simulink model "PV_Source_shading"  (R2025b)
settings: Solver=FixedStepDiscrete  StartTime=0.0  StopTime=0.5  FixedStep=Ts  RelTol=1e-3
InitFcn:
  | Ts = 1e-06;
libraries: spsSeriesRLCBranchLib x4, spsDiodeLib x3, spsPVArrayLib x2, spsVoltageMeasurementLib x2, simulink x1, spsCurrentMeasurementLib x1, spsIdealSwitchLib x1, spsDCVoltageSourceLib x1, spspowerguiLib x1
settings Model: Creator=JESHNU PRANAV  LastModifiedBy=JESHNU PRANAV
settings SolverCC: AutoInsertRateTranBlk=on

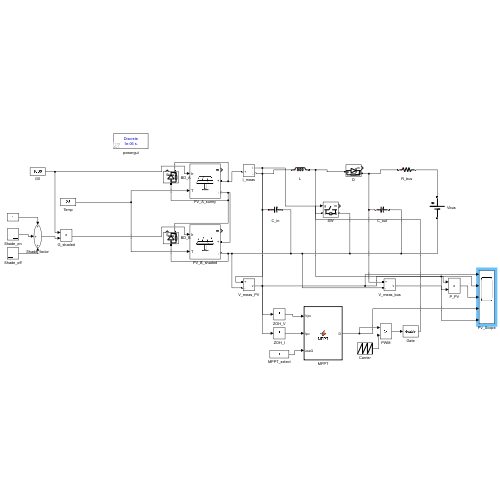
[thumbnail: Simulink's stored preview of the top-level diagram]
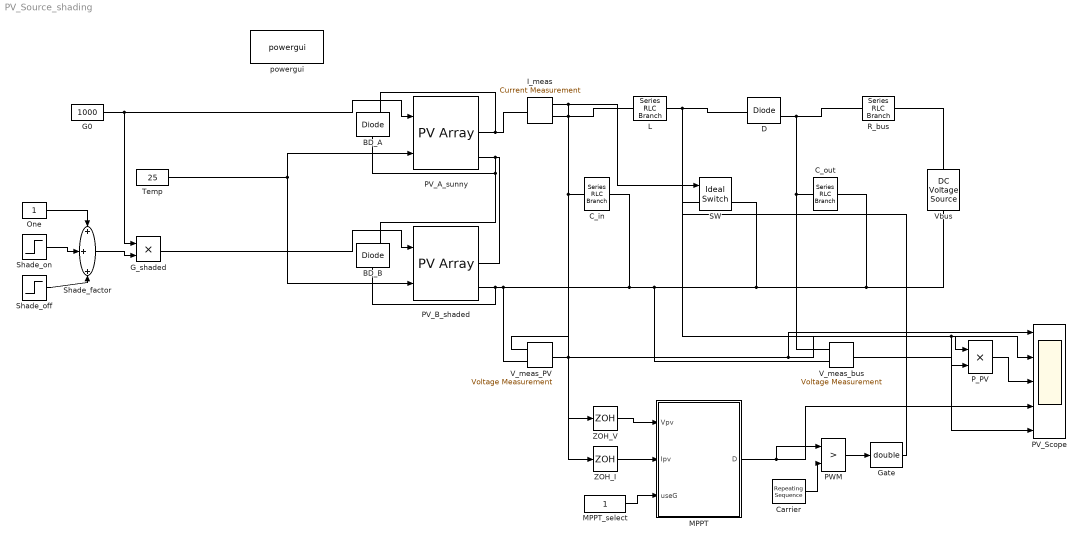
== system PV_Source_shading ==
  BD_A : spsDiodeLib/Diode  Ron=0.001  Lon=0  Vf=0.8  IC=0  UseSnubber=0  Rs=500  Cs=250e-9  Measurements=on
  BD_B : spsDiodeLib/Diode  Ron=0.001  Lon=0  Vf=0.8  IC=0  UseSnubber=0  Rs=500  Cs=250e-9  Measurements=on
  C_in : spsSeriesRLCBranchLib/Series RLC Branch  LConnTagsString=__new0  RConnTagsString=__new0  BranchType=C  Resistance=1  Inductance=1e-3  SetiL0=off  InitialCurrent=0  Capacitance=270e-6  Setx0=off  InitialVoltage=0  Measurements=None
  C_out : spsSeriesRLCBranchLib/Series RLC Branch  LConnTagsString=__new0  RConnTagsString=__new0  BranchType=C  Resistance=1  Inductance=1e-3  SetiL0=off  InitialCurrent=0  Capacitance=270e-6  Setx0=off  InitialVoltage=0  Measurements=None
  Carrier : simulink/Sources/Repeating Sequence  rep_seq_t=[0 5e-05]  rep_seq_y=[0 1]
  D : spsDiodeLib/Diode  Ron=0.001  Lon=0  Vf=0.8  IC=0  UseSnubber=0  Rs=500  Cs=250e-9  Measurements=on
  G0 : Constant  Value=1000
  G_shaded : Product
  Gate : DataTypeConversion  OutDataTypeStr=double  SaturateOnIntegerOverflow=off  RndMeth=Floor
  I_meas : spsCurrentMeasurementLib/Current Measurement  PhasorSimulation=off  OutputType=Complex  PSBequivalent=0
  L : spsSeriesRLCBranchLib/Series RLC Branch  LConnTagsString=__new0  RConnTagsString=__new0  BranchType=L  Resistance=1  Inductance=0.30e-3  SetiL0=off  InitialCurrent=0  Capacitance=1e-6  Setx0=off  InitialVoltage=0  Measurements=None
  MPPT : MATLAB Function  TreatAsAtomicUnit=on
  MPPT_select : Constant
  One : Constant
  PV_A_sunny : spsPVArrayLib/PV Array  Npar=8  Nser=4  PlotType=array @ 1000 W/m2 & specified temperatures  S_vec="[ 1000  500  100 ]"  Temp_C_vec="[ 45 25  ]"  ModuleName=User-defined  PlotWhenSelected=off  Pm=400  Ncell=72  Voc=48  Isc=10.5  Vm=40  Im=10  beta_Voc_pc=-0.36099  alpha_Isc_pc=0.102  beta_Voc=-0.17328  alpha_Isc=0.01071  IL=10.576  I0=3.9433e-10  nI=1.0809  Rsh=821.7644  Rs=0.20021  RobustModel=off  RobustCellTemperature=313.3991  BAL=on  Tc=1e-6  Tfilter=5e-5
  PV_B_shaded : spsPVArrayLib/PV Array  Npar=8  Nser=2  PlotType=array @ 1000 W/m2 & specified temperatures  S_vec="[ 1000  500  100 ]"  Temp_C_vec="[ 45 25  ]"  ModuleName=User-defined  PlotWhenSelected=off  Pm=400  Ncell=72  Voc=48  Isc=10.5  Vm=40  Im=10  beta_Voc_pc=-0.36099  alpha_Isc_pc=0.102  beta_Voc=-0.17328  alpha_Isc=0.01071  IL=10.576  I0=3.9433e-10  nI=1.0809  Rsh=821.7644  Rs=0.20021  RobustModel=off  RobustCellTemperature=313.3991  BAL=on  Tc=1e-6  Tfilter=5e-5
  PV_Scope : Scope  NumInputPorts=5
      settings: ActiveDisplayYMinimum=-928.47453257571487  ActiveDisplayYMaximum=10931.455878760957  DataLoggingDecimation=20  DataLoggingVariableName=pvdata
  PWM : RelationalOperator  Operator=>  OutDataTypeStr=boolean  RndMeth=Simplest  InputSameDT=off
  P_PV : Product
  R_bus : spsSeriesRLCBranchLib/Series RLC Branch  LConnTagsString=__new0  RConnTagsString=__new0  BranchType=R  Resistance=0.1  Inductance=1e-3  SetiL0=off  InitialCurrent=0  Capacitance=1e-6  Setx0=off  InitialVoltage=0  Measurements=None
  SW : spsIdealSwitchLib/Ideal Switch  Ron=0.001  Lon=0  IC=0  Rs=1e5  Cs=inf  Measurements=on
  Shade_factor : Sum  Inputs=+++
  Shade_off : Step  Time=0.35  After=0.7  SampleTime=0
  Shade_on : Step  Time=0.15  After=-0.7  SampleTime=0
  Temp : Constant  Value=25
  V_meas_PV : spsVoltageMeasurementLib/Voltage Measurement  PhasorSimulation=off  OutputType=Complex  PSBequivalent=0
  V_meas_bus : spsVoltageMeasurementLib/Voltage Measurement  PhasorSimulation=off  OutputType=Complex  PSBequivalent=0
  Vbus : spsDCVoltageSourceLib/DC Voltage Source  Amplitude=400  Measurements=None
  ZOH_I : ZeroOrderHold  SampleTime=0.0001
  ZOH_V : ZeroOrderHold  SampleTime=0.0001
  powergui : spspowerguiLib/powergui  Priority=1  SimulationMode=Discrete  SampleTime=Ts  frequency=60  Iterations=50  frequencyindice=0  Pbase=100e6  ErrMax=1e-4  UnitsV=kV  UnitsW=MW  buscounter=0  FunctionMessages=off  echomessages=off  EnableUseOfTLC=off  CurrentSourceSwitches=off  DisableSnubberDevices=off  DisableRonSwitches=off  DisableVfSwitches=off  DisplayEquations=off  AutomaticDiscreteSolvers=off  SolverType=Tustin/Backward Euler (TBE)  Interpol=off  ExternalGateDelay=off  methode=off  Ts=100  x0status=blocks  SPID=on  SwTol=0  HookPort=off  NonlinearTolerance=1e-4  nMaxIteration=100  ContinueOnMaxIteration=off  RestoreLinks=warning  ResistiveCurrentMeasurement=off  Frange=[0:2:500]  Ylog=off  Xlog=on  ShowGrid=off  save=off  variable=ZData  structure=0  ZoomFFT=off  StartTime=0.0  cycles=1  DisplayStyle=1  fundamental=60  FreqAxis=off  MaxFrequency=1000  frequencyindicesteady=1  RmsSteady=1  display=off
  wires:
  One/1 -> Shade_factor/1
  Shade_on/1 -> Shade_factor/2
  Shade_off/1 -> Shade_factor/3
  G0/1 -> G_shaded/1, PV_A_sunny/1
  Shade_factor/1 -> G_shaded/2
  G_shaded/1 -> PV_B_shaded/1
  Temp/1 -> PV_A_sunny/2, PV_B_shaded/2
  V_meas_PV/1 -> P_PV/1, PV_Scope/1, ZOH_V/1
  I_meas/1 -> P_PV/2, PV_Scope/2, ZOH_I/1
  ZOH_V/1 -> MPPT/1(Vpv)
  ZOH_I/1 -> MPPT/2(Ipv)
  MPPT_select/1 -> MPPT/3(useG)
  MPPT/1(D) -> PWM/1, PV_Scope/4
  Carrier/1 -> PWM/2
  PWM/1 -> Gate/1
  Gate/1 -> SW/1
  P_PV/1 -> PV_Scope/3
  V_meas_bus/1 -> PV_Scope/5
  connections:
  I_meas/LConn1 -- PV_A_sunny/RConn1 -- BD_A/RConn1
  PV_B_shaded/RConn1 -- PV_A_sunny/RConn2 -- BD_A/LConn1 -- BD_B/RConn1
  C_in/LConn1 -- I_meas/RConn1 -- L/LConn1 -- V_meas_PV/LConn1
  SW/LConn1 -- L/RConn1 -- D/LConn1
  C_out/LConn1 -- D/RConn1 -- R_bus/LConn1 -- V_meas_bus/LConn1
  R_bus/RConn1 -- Vbus/RConn1
  BD_B/LConn1 -- PV_B_shaded/RConn2 -- C_out/RConn1 -- Vbus/LConn1 -- SW/RConn1 -- V_meas_bus/LConn2 -- C_in/RConn1 -- V_meas_PV/LConn2

== matlab function PV_Source_shading/MPPT ==
  data: Vpv input; D output; Ipv input; useG input
function D = MPPT(Vpv, Ipv, useG)
% useG = 0 : standard P&O
% useG = 1 : Global MPPT = event-triggered full scan + P&O
% Boost on a 400 V bus: Vpv = (1 - D)*400, lowering D raises Vpv.
persistent mstate Dold Vold Pold k Dbest Pbest Pref holdc Psum
if isempty(mstate)
    Vold = 0; Pold = 0; k = 0; Pbest = 0; Pref = 0; holdc = 0; Psum = 0;
    if useG > 0.5, mstate = 1; Dold = 0.70; Dbest = 0.70;
    else,          mstate = 0; Dold = 0.40; Dbest = 0.40; end
end
dD = 0.002;  P = Vpv*Ipv;

if useG < 0.5   % ---------- standard P&O ----------
    dV = Vpv - Vold;  dP = P - Pold;
    if dP == 0, D = Dold; elseif dP*dV > 0, D = Dold - dD; else, D = Dold + dD; end
    D = min(max(D, 0.05), 0.85);
    Vold = Vpv; Pold = P; Dold = D;
    return
end

% ---------- Global MPPT ----------
Dlo = 0.30; Dhi = 0.70;      % scan range: Vpv = 280 V ... 120 V
dscan = 0.025; nset = 40; navg = 10;   % 17 points x 4 ms = ~70 ms scan
if mstate == 1               % SCAN: step D, wait to settle, record power
    k = k + 1;
    if k > nset - navg, Psum = Psum + P; end
    if k >= nset
        Pm = Psum/navg;
        if Pm > Pbest, Pbest = Pm; Dbest = Dold; end
        k = 0; Psum = 0;
        D = Dold - dscan;
        if D < Dlo - 1e-9     % scan done: jump to the best (global) point
            D = Dbest; mstate = 0; Pref = Pbest; holdc = 300;
        end
    else
        D = Dold;
    end
    Vold = Vpv; Pold = P; Dold = D;
    return
end
% P&O around the global peak
dV = Vpv - Vold;  dP = P - Pold;
if dP == 0, D = Dold; elseif dP*dV > 0, D = Dold - dD; else, D = Dold + dD; end
D = min(max(D, Dlo), Dhi);
if holdc > 0
    holdc = holdc - 1;
elseif Pref > 0 && abs(P - Pref) > 0.15*Pref   % sudden change (shading) -> rescan
    mstate = 1; k = 0; Psum = 0; Pbest = 0; D = Dhi;
else
    Pref = 0.995*Pref + 0.005*P;               % follow slow changes
end
Vold = Vpv; Pold = P; Dold = D;
